simulink subsystem "Human_Input_Pre_Processing_sub"  (R2023b)
settings: Solver=VariableStepAuto  StartTime=0.0  StopTime=10.0  RelTol=1e-3
libraries: simulink x19
settings Model: Creator=ander  LastModifiedBy=ander

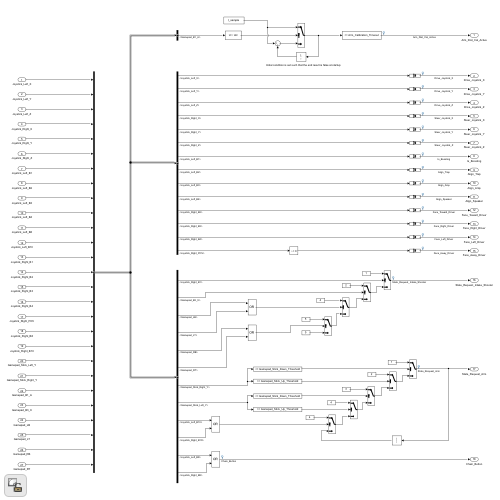
[thumbnail: Simulink's stored preview of the top-level diagram]
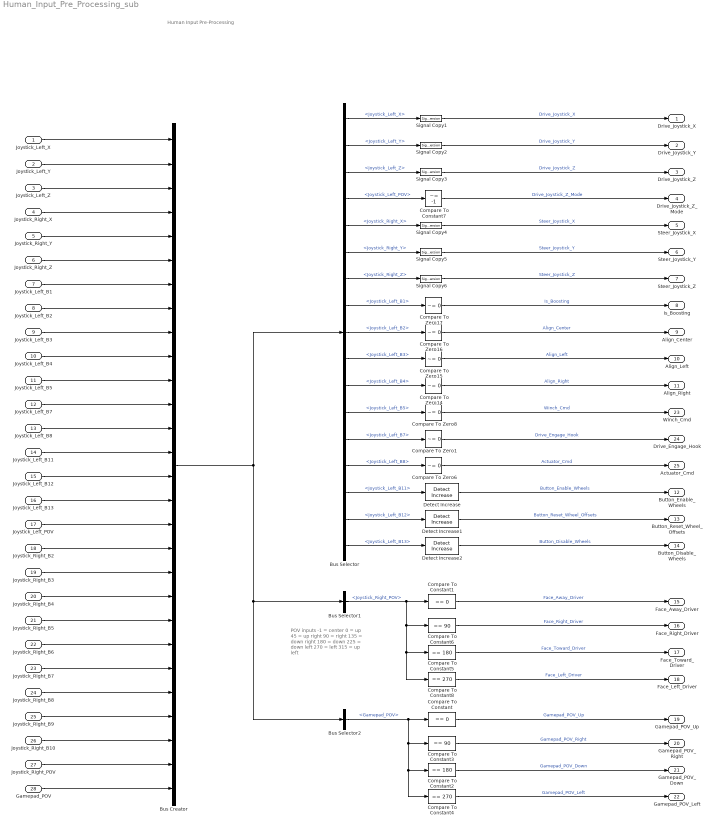
== system Human_Input_Pre_Processing_sub ==
  note: POV inputs
      | -1 = center
      | 0 = up
      | 45 = up right
      | 90 = right
      | 135 = down right
      | 180 = down
      | 225 = down left
      | 270 = left
      | 315 = up left
  note: Human Input Pre-Processing
  Joystick_Left_X : Inport
  Joystick_Left_Y : Inport  Port=2
  Joystick_Left_Z : Inport  Port=3
  Joystick_Right_X : Inport  Port=4
  Joystick_Right_Y : Inport  Port=5
  Joystick_Right_Z : Inport  Port=6
  Joystick_Left_B1 : Inport  Port=7
  Joystick_Left_B2 : Inport  Port=8
  Joystick_Left_B3 : Inport  Port=9
  Joystick_Left_B4 : Inport  Port=10
  Joystick_Left_B5 : Inport  Port=11
  Joystick_Left_B7 : Inport  Port=12
  Joystick_Left_B8 : Inport  Port=13
  Joystick_Left_B11 : Inport  Port=14
  Joystick_Left_B12 : Inport  Port=15
  Joystick_Left_B13 : Inport  Port=16
  Joystick_Left_POV : Inport  Port=17
  Joystick_Right_B2 : Inport  Port=18
  Joystick_Right_B3 : Inport  Port=19
  Joystick_Right_B4 : Inport  Port=20
  Joystick_Right_B5 : Inport  Port=21
  Joystick_Right_B6 : Inport  Port=22
  Joystick_Right_B7 : Inport  Port=23
  Joystick_Right_B8 : Inport  Port=24
  Joystick_Right_B9 : Inport  Port=25
  Joystick_Right_B10 : Inport  Port=26
  Joystick_Right_POV : Inport  Port=27
  Gamepad_POV : Inport  Port=28
  Bus Creator : BusCreator  Inputs=28
  Bus Selector : BusSelector  OutputSignals=Joystick_Left_X,Joystick_Left_Y,Joystick_Left_Z,Joystick_Left_POV,Joystick_Right_X,Joystick_Right_Y,Joystick_Right_Z,Joystick_Left_B1,Joystick_Left_B2,Joystick_Left_B3,Joystick_Left_B4,Joystick_Left_B5,Joystick_Left_B7,Joystick_Left_B8,Joystick_Left_B11,Joystick_Left_B12,Joystick_Left_B13
  Bus Selector1 : BusSelector  OutputSignals=Joystick_Right_POV
  Bus Selector2 : BusSelector  OutputSignals=Gamepad_POV
  Compare To Constant : simulink/Logic and Bit Operations/Compare To Constant  relop===  const=0  OutDataTypeStr=boolean
  Compare To Constant1 : simulink/Logic and Bit Operations/Compare To Constant  relop===  const=0  OutDataTypeStr=boolean
  Compare To Constant2 : simulink/Logic and Bit Operations/Compare To Constant  relop===  const=180  OutDataTypeStr=boolean
  Compare To Constant3 : simulink/Logic and Bit Operations/Compare To Constant  relop===  const=90  OutDataTypeStr=boolean
  Compare To Constant4 : simulink/Logic and Bit Operations/Compare To Constant  relop===  const=270  OutDataTypeStr=boolean
  Compare To Constant5 : simulink/Logic and Bit Operations/Compare To Constant  relop===  const=180  OutDataTypeStr=boolean
  Compare To Constant6 : simulink/Logic and Bit Operations/Compare To Constant  relop===  const=90  OutDataTypeStr=boolean
  Compare To Constant7 : simulink/Logic and Bit Operations/Compare To Constant  relop=~=  const=-1  OutDataTypeStr=boolean
  Compare To Constant8 : simulink/Logic and Bit Operations/Compare To Constant  relop===  const=270  OutDataTypeStr=boolean
  Compare To Zero{1,6,8,14..17} (7 alike) : simulink/Logic and Bit Operations/Compare To Zero  relop=~=  OutDataTypeStr=boolean
  Detect Increase : simulink/Logic and Bit Operations/Detect Increase  vinit=0.0  OutDataTypeStr=boolean
  Detect Increase1 : simulink/Logic and Bit Operations/Detect Increase  vinit=0.0  OutDataTypeStr=boolean
  Detect Increase2 : simulink/Logic and Bit Operations/Detect Increase  vinit=0.0  OutDataTypeStr=boolean
  Signal Copy{1..6} (6 alike) : SignalConversion  OverrideOpt=off
  Drive_Joystick_X : Outport
  Drive_Joystick_Y : Outport  Port=2
  Drive_Joystick_Z : Outport  Port=3
  Drive_Joystick_Z_Mode : Outport  Port=4
  Steer_Joystick_X : Outport  Port=5
  Steer_Joystick_Y : Outport  Port=6
  Steer_Joystick_Z : Outport  Port=7
  Is_Boosting : Outport  Port=8
  Align_Center : Outport  Port=9
  Align_Left : Outport  Port=10
  Align_Right : Outport  Port=11
  Button_Enable_Wheels : Outport  Port=12
  Button_Reset_Wheel_Offsets : Outport  Port=13
  Button_Disable_Wheels : Outport  Port=14
  Face_Away_Driver : Outport  Port=15
  Face_Right_Driver : Outport  Port=16
  Face_Toward_Driver : Outport  Port=17
  Face_Left_Driver : Outport  Port=18
  Gamepad_POV_Up : Outport  Port=19
  Gamepad_POV_Right : Outport  Port=20
  Gamepad_POV_Down : Outport  Port=21
  Gamepad_POV_Left : Outport  Port=22
  Winch_Cmd : Outport  Port=23
  Drive_Engage_Hook : Outport  Port=24
  Actuator_Cmd : Outport  Port=25
  wires:
  Bus Creator/1 -> Bus Selector1/1, Bus Selector2/1, Bus Selector/1
  Signal Copy1/1 -> Drive_Joystick_X/1  "Drive_Joystick_X"
  Signal Copy6/1 -> Steer_Joystick_Z/1  "Steer_Joystick_Z"
  Signal Copy5/1 -> Steer_Joystick_Y/1  "Steer_Joystick_Y"
  Signal Copy4/1 -> Steer_Joystick_X/1  "Steer_Joystick_X"
  Signal Copy3/1 -> Drive_Joystick_Z/1  "Drive_Joystick_Z"
  Signal Copy2/1 -> Drive_Joystick_Y/1  "Drive_Joystick_Y"
  Compare To Zero14/1 -> Align_Right/1  "Align_Right"
  Compare To Zero17/1 -> Is_Boosting/1  "Is_Boosting"
  Compare To Constant7/1 -> Drive_Joystick_Z_Mode/1  "Drive_Joystick_Z_Mode"
  Bus Selector/1 -> Signal Copy1/1  "<Joystick_Left_X>"
  Bus Selector/2 -> Signal Copy2/1  "<Joystick_Left_Y>"
  Bus Selector/3 -> Signal Copy3/1  "<Joystick_Left_Z>"
  Bus Selector/4 -> Compare To Constant7/1  "<Joystick_Left_POV>"
  Bus Selector/5 -> Signal Copy4/1  "<Joystick_Right_X>"
  Bus Selector/6 -> Signal Copy5/1  "<Joystick_Right_Y>"
  Bus Selector/7 -> Signal Copy6/1  "<Joystick_Right_Z>"
  Bus Selector/9 -> Compare To Zero16/1  "<Joystick_Left_B2>"
  Bus Selector/8 -> Compare To Zero17/1  "<Joystick_Left_B1>"
  Bus Selector/10 -> Compare To Zero15/1  "<Joystick_Left_B3>"
  Bus Selector/11 -> Compare To Zero14/1  "<Joystick_Left_B4>"
  Joystick_Left_X/1 -> Bus Creator/1
  Joystick_Left_Y/1 -> Bus Creator/2
  Joystick_Left_Z/1 -> Bus Creator/3
  Joystick_Right_X/1 -> Bus Creator/4
  Joystick_Right_Y/1 -> Bus Creator/5
  Joystick_Right_Z/1 -> Bus Creator/6
  Joystick_Left_B1/1 -> Bus Creator/7
  Joystick_Left_B2/1 -> Bus Creator/8
  Joystick_Left_B3/1 -> Bus Creator/9
  Joystick_Left_B4/1 -> Bus Creator/10
  Bus Selector/15 -> Detect Increase/1  "<Joystick_Left_B11>"
  Bus Selector/16 -> Detect Increase1/1  "<Joystick_Left_B12>"
  Bus Selector/17 -> Detect Increase2/1  "<Joystick_Left_B13>"
  Detect Increase/1 -> Button_Enable_Wheels/1  "Button_Enable_Wheels"
  Detect Increase1/1 -> Button_Reset_Wheel_Offsets/1  "Button_Reset_Wheel_Offsets"
  Detect Increase2/1 -> Button_Disable_Wheels/1  "Button_Disable_Wheels"
  Compare To Constant/1 -> Gamepad_POV_Up/1  "Gamepad_POV_Up"
  Compare To Constant2/1 -> Gamepad_POV_Down/1  "Gamepad_POV_Down"
  Compare To Constant3/1 -> Gamepad_POV_Right/1  "Gamepad_POV_Right"
  Compare To Constant4/1 -> Gamepad_POV_Left/1  "Gamepad_POV_Left"
  Compare To Zero15/1 -> Align_Left/1  "Align_Left"
  Compare To Zero16/1 -> Align_Center/1  "Align_Center"
  Bus Selector1/1 -> Compare To Constant1/1, Compare To Constant6/1, Compare To Constant5/1, Compare To Constant8/1  "<Joystick_Right_POV>"
  Bus Selector2/1 -> Compare To Constant/1, Compare To Constant3/1, Compare To Constant2/1, Compare To Constant4/1  "<Gamepad_POV>"
  Compare To Constant1/1 -> Face_Away_Driver/1  "Face_Away_Driver"
  Compare To Constant6/1 -> Face_Right_Driver/1  "Face_Right_Driver"
  Compare To Constant5/1 -> Face_Toward_Driver/1  "Face_Toward_Driver"
  Compare To Constant8/1 -> Face_Left_Driver/1  "Face_Left_Driver"
  Joystick_Left_B5/1 -> Bus Creator/11
  Joystick_Left_B7/1 -> Bus Creator/12
  Joystick_Left_B8/1 -> Bus Creator/13
  Joystick_Left_B11/1 -> Bus Creator/14
  Joystick_Left_B12/1 -> Bus Creator/15
  Joystick_Left_B13/1 -> Bus Creator/16
  Joystick_Left_POV/1 -> Bus Creator/17
  Joystick_Right_B2/1 -> Bus Creator/18
  Joystick_Right_B3/1 -> Bus Creator/19
  Joystick_Right_B4/1 -> Bus Creator/20
  Joystick_Right_B5/1 -> Bus Creator/21
  Joystick_Right_B6/1 -> Bus Creator/22
  Joystick_Right_B7/1 -> Bus Creator/23
  Joystick_Right_B8/1 -> Bus Creator/24
  Joystick_Right_B9/1 -> Bus Creator/25
  Joystick_Right_B10/1 -> Bus Creator/26
  Joystick_Right_POV/1 -> Bus Creator/27
  Gamepad_POV/1 -> Bus Creator/28
  Compare To Zero8/1 -> Winch_Cmd/1  "Winch_Cmd"
  Bus Selector/12 -> Compare To Zero8/1  "<Joystick_Left_B5>"
  Bus Selector/14 -> Compare To Zero6/1  "<Joystick_Left_B8>"
  Compare To Zero6/1 -> Actuator_Cmd/1  "Actuator_Cmd"
  Bus Selector/13 -> Compare To Zero1/1  "<Joystick_Left_B7>"
  Compare To Zero1/1 -> Drive_Engage_Hook/1  "Drive_Engage_Hook"
